simulink model "UAV3_MissionLifecycle"  (R2026b)
settings: Solver=FixedStepDiscrete  FixedStep=0.1
settings Model: Creator=Ivan  LastModifiedBy=Ivan

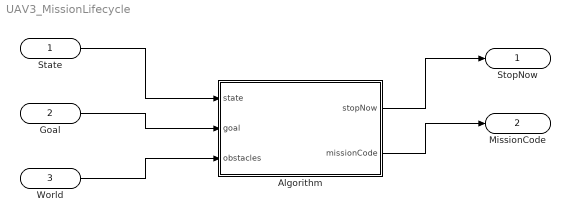
== system UAV3_MissionLifecycle ==
  State : Inport  OutDataTypeStr=double  PortDimensions=[5 1]
  Goal : Inport  Port=2  OutDataTypeStr=double  PortDimensions=[2 1]
  World : Inport  Port=3  OutDataTypeStr=double  PortDimensions=[3 2]
  Algorithm : MATLAB Function  TreatAsAtomicUnit=on
  StopNow : Outport
  MissionCode : Outport  Port=2
  wires:
  State/1 -> Algorithm/1(state)
  Goal/1 -> Algorithm/2(goal)
  World/1 -> Algorithm/3(obstacles)
  Algorithm/1(stopNow) -> StopNow/1
  Algorithm/2(missionCode) -> MissionCode/1

== matlab function UAV3_MissionLifecycle/Algorithm ==
  data: state input; stopNow output; goal input; obstacles input; missionCode output
function [stopNow, missionCode] = mission_supervisor(state, goal, obstacles)
%MISSION_SUPERVISOR Terminal state machine for 2D training simulation.
% state [x;y;vx;vy;battery]; goal [x;y]; obstacles [3xN].
% Codes: 0=FLYING, 1=GOAL_REACHED, 2=COLLISION,
%        3=LOW_BATTERY, 4=INVALID_STATE.
%#codegen
missionCode = 0;
stopNow = false;

if any(~isfinite(state)) || any(~isfinite(goal))
    missionCode = 4;
    stopNow = true;
    return;
end

% Collision has priority over goal arrival (no false success on collision).
for k = 1:size(obstacles,2)
    if norm(state(1:2)-obstacles(1:2,k)) <= obstacles(3,k)
        missionCode = 2;
        stopNow = true;
        return;
    end
end

if state(5) <= 5.0
    missionCode = 3;
    stopNow = true;
    return;
end

distanceToGoal = norm(state(1:2)-goal);
speed = norm(state(3:4));
if distanceToGoal <= 3.0 && speed <= 1.0
    missionCode = 1;
    stopNow = true;
end
end
